simulink model "Sistema_completo"  (R2026b)
settings: Solver=FixedStepAuto  StopTime=Tsim  FixedStep=Ts
InitFcn:
  | sys_params
values from neighbouring files (symbols this model uses):
  D = 20    [sys_params.m]    (also in sys_params_original.m)
  fLO = fc_rx + fIF    (= 2340000)    [sys_params.m]    (also in sys_params_original.m)
  fm = [2e3 5e3 10e3]    [sys_params.m]
  fsub = P('fsub')    [radio_gui.m]    (also in radio_guiV2.m; sys_params.m = [fc1 fc2 fc3]; sys_params_original.m = [20e3 60e3 100e3])
  K_FDM = 1/3    (= 0.333333333333)    [sys_params.m]    (also in sys_params_original.m)
  L = Fs/Fs_tx    (= 40)    [sys_params.m]
  noiseVar = Pc*(Fs/2)/(10^(CNRdB/10)*BT)    [sys_params.m]
  phi = -2*pi*fsub*tau    [calibrate.m]    (also in phi.mat = [-6.55022068273 -7.86026481928 -10.0436717135]; sys_params.m = zeros(1,3); sys_params_original.m = zeros(1,3))
  Ts = 1/Fs    (= 5e-08)    [sys_params.m]    (also in sys_params_original.m = 2e-06)
  Ts2 = 1/Fs2    (= 1e-06)    [sys_params.m]    (also in sys_params_original.m = 4e-05)
  Ts_tx = 1/Fs_tx    (= 2e-06)    [sys_params.m]
undefined symbols (not defined in the file or in its folder): designMultirateFIR
libraries: dsparch4 x7, commanapbnd3 x5, dspmlti4 x2, dspfdesign x1
settings Model: SimulationMode=accelerator  Creator=felipe  LastModifiedBy=matia

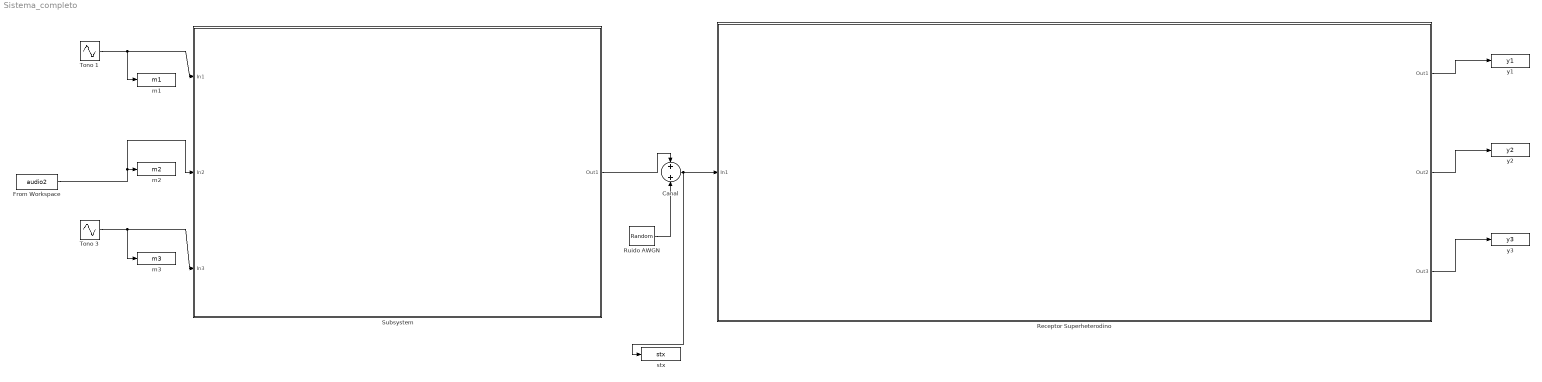
== system Sistema_completo ==
  Canal : Sum
  From Workspace : FromWorkspace  VariableName=audio2  SampleTime=Ts_tx  Interpolate=off  OutputAfterFinalValue=Setting to zero
  Receptor Superheterodino : Subsystem
  Ruido AWGN : RandomNumber  Variance=noiseVar  Seed=12345  SampleTime=Ts
  Subsystem : Subsystem
  Tono 1 : Sin  Frequency=2*pi*fm(1)  SampleTime=Ts_tx
  Tono 3 : Sin  Frequency=2*pi*fm(3)  SampleTime=Ts_tx
  m1 : ToWorkspace  VariableName=m1  SampleTime=-1
  m2 : ToWorkspace  VariableName=m2  SampleTime=-1
  m3 : ToWorkspace  VariableName=m3  SampleTime=-1
  stx : ToWorkspace  VariableName=stx  SampleTime=-1
      settings: MaxDataPoints=2^18
  y1 : ToWorkspace  VariableName=y1  SampleTime=-1
  y2 : ToWorkspace  VariableName=y2  SampleTime=-1
  y3 : ToWorkspace  VariableName=y3  SampleTime=-1
  wires:
  Tono 1/1 -> Subsystem/1(In1), m1/1
  Receptor Superheterodino/1(Out1) -> y1/1
  From Workspace/1 -> Subsystem/2(In2), m2/1
  Receptor Superheterodino/2(Out2) -> y2/1
  Tono 3/1 -> Subsystem/3(In3), m3/1
  Receptor Superheterodino/3(Out3) -> y3/1
  Subsystem/1(Out1) -> Canal/1
  Ruido AWGN/1 -> Canal/2
  Canal/1 -> Receptor Superheterodino/1(In1), stx/1

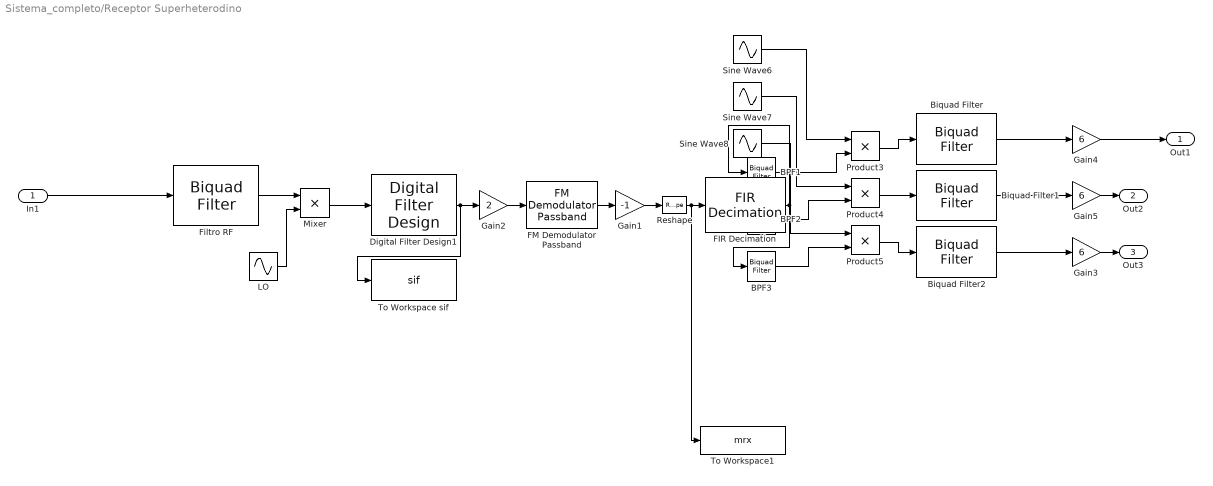
== system Sistema_completo/Receptor Superheterodino ==
  In1 : Inport
  BPF1 : dsparch4/Biquad Filter  FilterSource=Dialog parameters  CoeffSource=Specify via dialog  FilterObject=BQF  IIRFiltStruct=Direct form II transposed  BiQuadCoeffs=sosBP1  ScaleValues=1  IC=0  ICnum=0  ICden=0  a0Flag=Warning  optimizeScaleValues=on  ScaleValueMode=Specify via input port (g)  roundingMode=Floor  overflowMode=off  scaleValueFracLength=14  denProdOutputFracLength=30  denAccumFracLength=30  secondMemoryFracLength=15
  BPF2 : dsparch4/Biquad Filter  FilterSource=Dialog parameters  CoeffSource=Specify via dialog  FilterObject=BQF  IIRFiltStruct=Direct form II transposed  BiQuadCoeffs=sosBP2  ScaleValues=1  IC=0  ICnum=0  ICden=0  a0Flag=Warning  optimizeScaleValues=on  ScaleValueMode=Specify via input port (g)  roundingMode=Floor  overflowMode=off  scaleValueFracLength=14  denProdOutputFracLength=30  denAccumFracLength=30  secondMemoryFracLength=15
  BPF3 : dsparch4/Biquad Filter  FilterSource=Dialog parameters  CoeffSource=Specify via dialog  FilterObject=BQF  IIRFiltStruct=Direct form II transposed  BiQuadCoeffs=sosBP3  ScaleValues=1  IC=0  ICnum=0  ICden=0  a0Flag=Warning  optimizeScaleValues=on  ScaleValueMode=Specify via input port (g)  roundingMode=Floor  overflowMode=off  scaleValueFracLength=14  denProdOutputFracLength=30  denAccumFracLength=30  secondMemoryFracLength=15
  Biquad Filter : dsparch4/Biquad Filter  FilterSource=Dialog parameters  CoeffSource=Specify via dialog  FilterObject=BQF  IIRFiltStruct=Direct form II transposed  BiQuadCoeffs=sosAud1  ScaleValues=1  IC=0  ICnum=0  ICden=0  a0Flag=Warning  optimizeScaleValues=on  ScaleValueMode=Specify via input port (g)  InputProcessing=Columns as channels (frame based)  roundingMode=Floor  overflowMode=off  scaleValueFracLength=14  denProdOutputFracLength=30  denAccumFracLength=30  secondMemoryFracLength=15
  Biquad Filter1 : dsparch4/Biquad Filter  FilterSource=Dialog parameters  CoeffSource=Specify via dialog  FilterObject=BQF  IIRFiltStruct=Direct form II transposed  BiQuadCoeffs=sosAud2  ScaleValues=1  IC=0  ICnum=0  ICden=0  a0Flag=Warning  optimizeScaleValues=on  ScaleValueMode=Specify via input port (g)  InputProcessing=Columns as channels (frame based)  roundingMode=Floor  overflowMode=off  scaleValueFracLength=14  denProdOutputFracLength=30  denAccumFracLength=30  secondMemoryFracLength=15
  Biquad Filter2 : dsparch4/Biquad Filter  FilterSource=Dialog parameters  CoeffSource=Specify via dialog  FilterObject=BQF  IIRFiltStruct=Direct form II transposed  BiQuadCoeffs=sosAud3  ScaleValues=1  IC=0  ICnum=0  ICden=0  a0Flag=Warning  optimizeScaleValues=on  ScaleValueMode=Specify via input port (g)  InputProcessing=Columns as channels (frame based)  roundingMode=Floor  overflowMode=off  scaleValueFracLength=14  denProdOutputFracLength=30  denAccumFracLength=30  secondMemoryFracLength=15
  Digital Filter Design1 : dspfdesign/Digital Filter Design  mwdsp_browser_bugfix_var=off
  FIR Decimation : dspmlti4/FIR Decimation  FilterSource=Dialog parameters  h=hDec  D=D  filtStruct=Direct form  FilterObject=FDECIM  framing=Enforce single-rate processing  AllowArbitraryInputLength=off  inputOffset=0  outputBufInitCond=0  roundingMode=Floor  overflowMode=off  firstCoeffDataTypeStr=Inherit: Same word length as input  firstCoeffMin=[]  firstCoeffMax=[]  firstCoeffLastDataTypeStr=Inherit: Same word length as input  outputDataTypeStr=Inherit: Same as accumulator  outputMin=[]  outputMax=[]  outputLastDataTypeStr=Inherit: Same as accumulator
  FM Demodulator Passband : commanapbnd3/FM Demodulator Passband  Fc=fIF  Ph=0  Kc=df  Ho=1000
  Filtro RF : dsparch4/Biquad Filter  FilterSource=Dialog parameters  CoeffSource=Specify via dialog  FilterObject=BQF  IIRFiltStruct=Direct form II transposed  BiQuadCoeffs=sosRF  ScaleValues=1  IC=0  ICnum=0  ICden=0  a0Flag=Warning  optimizeScaleValues=on  ScaleValueMode=Specify via input port (g)  roundingMode=Floor  overflowMode=off  scaleValueFracLength=14  denProdOutputFracLength=30  denAccumFracLength=30  secondMemoryFracLength=15
  Gain1 : Gain  Gain=-1
  Gain2 : Gain  Gain=2
  Gain3 : Gain  Gain=6
  Gain4 : Gain  Gain=6
  Gain5 : Gain  Gain=6
  LO : Sin  Frequency=2*pi*fLO  SampleTime=Ts
  Mixer : Product
  Product3 : Product
  Product4 : Product
  Product5 : Product
  Reshape : Reshape
  Sine Wave6 : Sin  Frequency=2*pi*fsub(1)  Phase=phi(1)  SampleTime=Ts2
  Sine Wave7 : Sin  Frequency=2*pi*fsub(2)  Phase=phi(2)  SampleTime=Ts2
  Sine Wave8 : Sin  Frequency=2*pi*fsub(3)  Phase=phi(3)  SampleTime=Ts2
  To Workspace sif : ToWorkspace  VariableName=sif  SampleTime=-1
      settings: MaxDataPoints=2^18
  To Workspace1 : ToWorkspace  VariableName=mrx  SampleTime=Ts
  Out1 : Outport
  Out2 : Outport  Port=2
  Out3 : Outport  Port=3
  wires:
  Gain3/1 -> Out3/1
  FM Demodulator Passband/1 -> Gain1/1
  Mixer/1 -> Digital Filter Design1/1
  Filtro RF/1 -> Mixer/1
  Gain4/1 -> Out1/1
  In1/1 -> Filtro RF/1
  Reshape/1 -> To Workspace1/1, FIR Decimation/1
  Sine Wave6/1 -> Product3/1
  Product3/1 -> Biquad Filter/1
  Gain2/1 -> FM Demodulator Passband/1
  Digital Filter Design1/1 -> Gain2/1, To Workspace sif/1
  Biquad Filter1/1 -> Gain5/1
  Biquad Filter2/1 -> Gain3/1
  Product4/1 -> Biquad Filter1/1
  Sine Wave8/1 -> Product5/1
  Product5/1 -> Biquad Filter2/1
  Biquad Filter/1 -> Gain4/1
  LO/1 -> Mixer/2
  Gain5/1 -> Out2/1
  Sine Wave7/1 -> Product4/1
  Gain1/1 -> Reshape/1
  FIR Decimation/1 -> BPF1/1, BPF2/1, BPF3/1
  BPF1/1 -> Product3/2
  BPF2/1 -> Product4/2
  BPF3/1 -> Product5/2

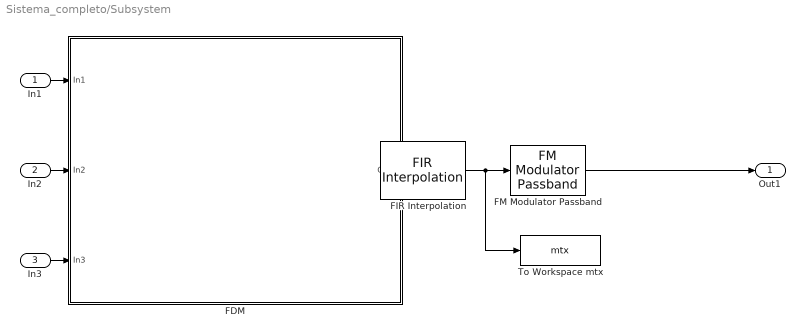
== system Sistema_completo/Subsystem ==
  In1 : Inport
  In2 : Inport  Port=2
  In3 : Inport  Port=3
  FDM : Subsystem
  FIR Interpolation : dspmlti4/FIR Interpolation  FilterSource=Auto  PrivateCoeffs=0  h=designMultirateFIR(L,1)  L=L  FilterObject=FINTERP  framing=Allow multirate processing  outputBufInitCond=0  roundingMode=Floor  overflowMode=off  firstCoeffDataTypeStr=Inherit: Same word length as input  firstCoeffMin=[]  firstCoeffMax=[]  firstCoeffLastDataTypeStr=Inherit: Same word length as input  outputMin=[]  outputMax=[]
  FM Modulator Passband : commanapbnd3/FM Modulator Passband  Fc=fc_tx  Ph=0  Kc=deltaf
  To Workspace mtx : ToWorkspace  VariableName=mtx  SampleTime=-1
  Out1 : Outport
  wires:
  In2/1 -> FDM/2(In2)
  In3/1 -> FDM/3(In3)
  In1/1 -> FDM/1(In1)
  FDM/1(Out1) -> FIR Interpolation/1
  FIR Interpolation/1 -> FM Modulator Passband/1, To Workspace mtx/1
  FM Modulator Passband/1 -> Out1/1

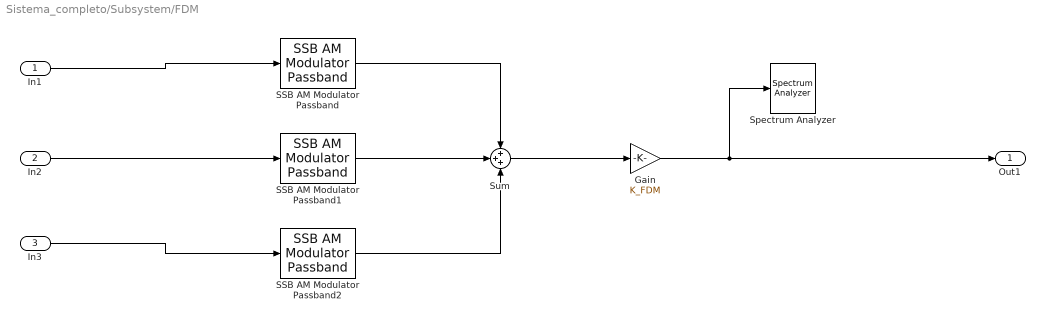
== system Sistema_completo/Subsystem/FDM ==
  In1 : Inport
  In2 : Inport  Port=2
  In3 : Inport  Port=3
  Gain : Gain  Gain=K_FDM
  SSB AM Modulator Passband : commanapbnd3/SSB AM Modulator Passband  Fc=fc1  Ph=0  Sd=Upper  Ho=Nh
  SSB AM Modulator Passband1 : commanapbnd3/SSB AM Modulator Passband  Fc=fc2  Ph=0  Sd=Upper  Ho=Nh
  SSB AM Modulator Passband2 : commanapbnd3/SSB AM Modulator Passband  Fc=fc3  Ph=0  Sd=Upper  Ho=Nh
  Spectrum Analyzer : SpectrumAnalyzer  WindowPosition=[375.000000,152.000000,800.000000,500.000000,]  Visible=on  ScopeFrameLocation=window  SampleRate=44.1e3  PlotAsTwoSidedSpectrum=off  AxesScaling=Manual  WindowInvariantSamplesPerUpdate=on  FrequencySpan=Start and stop frequencies  StartFrequency=0  StopFrequency=70e3  VBWSource=Property  VBW=10  MaximizeAxes=Off  PlotNormalTrace=off  PlotMaxHoldTrace=on  YLimits=[-70 49.3231]  SelectedToolstripTab=spectrumAnalyzerToolstrip.homeTab
      settings: OpenAtSimulationStart=off
  Sum : Sum  Inputs=+++
  Out1 : Outport
  wires:
  SSB AM Modulator Passband1/1 -> Sum/2
  SSB AM Modulator Passband2/1 -> Sum/3
  Sum/1 -> Gain/1
  SSB AM Modulator Passband/1 -> Sum/1
  Gain/1 -> Spectrum Analyzer/1, Out1/1
  In3/1 -> SSB AM Modulator Passband2/1
  In2/1 -> SSB AM Modulator Passband1/1
  In1/1 -> SSB AM Modulator Passband/1
